simulink model "PMSM_MC_2025a"  (R2025a)
settings: Solver=FixedStepDiscrete  StartTime=0.0  StopTime=10.0  FixedStep=0.00005  RelTol=1e-3
values from neighbouring files (symbols this model uses):
  MC_DCurrLopKi_CFG = 0.008293758    [PMSM_MC_Data_2025a.sldd]
  MC_DCurrLopKp_CFG = 0.0870848    [PMSM_MC_Data_2025a.sldd]
  MC_MotModeDebug_CFG = 255.0    [PMSM_MC_Data_2025a.sldd]
  MC_POLE_NUM_CFG = 7.0    [PMSM_MC_Data_2025a.sldd]
  MC_QCurrLopKi_CFG = 0.008293758    [PMSM_MC_Data_2025a.sldd]
  MC_QCurrLopKp_CFG = 0.0870848    [PMSM_MC_Data_2025a.sldd]
  MC_SpdLopKi_CFG = 1.0E-5    [PMSM_MC_Data_2025a.sldd]
  MC_SpdLopKp_CFG = 0.002    [PMSM_MC_Data_2025a.sldd]
  OpenLoopEn_CFG = 0.0    [PMSM_MC_Data_2025a.sldd]
  SensorLessEn_CFG = 0.0    [PMSM_MC_Data_2025a.sldd]
  SensorLessType_CFG = 1.0    [PMSM_MC_Data_2025a.sldd]
undefined symbols (not defined in the file or in its folder): Ls, magnitude, Rs
libraries: simulink x25, slpidlib x6
(part 2 of 3)

== system PMSM_MC_2025a/PMSM_MC/MC_HighFrqTask/FOC/SVPWM/SevenSegSVPWM ==
  Uα : Inport
  Uβ : Inport  Port=2
  VBus : Inport  Port=3
  Demux : Demux  Outputs=3
  SectorCaculate : Subsystem
  T1T2Caculate : Subsystem
  TcmCaculate : Subsystem
  Tpwm : Constant  Value=single(1)
  XYZCaculate : Subsystem
  UVoltage_PWM : Outport
  VVoltage_PWM : Outport  Port=2
  WVoltage_PWM : Outport  Port=3
  wires:
  Uα/1 -> SectorCaculate/1(Ualpha), XYZCaculate/1(Ualpha)
  Uβ/1 -> XYZCaculate/2(Ubeta), SectorCaculate/2(Ubeta)
  VBus/1 -> XYZCaculate/3(Udc)
  Tpwm/1 -> TcmCaculate/4(Tpwm), T1T2Caculate/3(Tpwm), XYZCaculate/4(Ts)
  SectorCaculate/1(N) -> TcmCaculate/1(N), T1T2Caculate/1(N)
  XYZCaculate/1(XYZ) -> T1T2Caculate/2(XYZ)
  T1T2Caculate/1(T1) -> TcmCaculate/2(T1)
  T1T2Caculate/2(T2) -> TcmCaculate/3(T2)
  TcmCaculate/1(Tcm1 Tcm2 Tcm3) -> Demux/1
  Demux/1 -> UVoltage_PWM/1
  Demux/2 -> VVoltage_PWM/1
  Demux/3 -> WVoltage_PWM/1

== system PMSM_MC_2025a/PMSM_MC/MC_HighFrqTask/FOC/SensorLessAlgorithm/FluxObs+PLL ==
  MotorSpdRef : Inport
  Ialpha : Inport  Port=2
  Ibeta : Inport  Port=3
  Ualpha : Inport  Port=4
  Ubeta : Inport  Port=5
  Enable : EnablePort
  FluxObs : Subsystem
  PLL : Subsystem
  Thetae_Est : Outport
  We_Est : Outport  Port=2
  wires:
  Ubeta/1 -> FluxObs/4(Ubeta)
  Ualpha/1 -> FluxObs/3(Ualpha)
  Ialpha/1 -> FluxObs/1(Ialpha)
  Ibeta/1 -> FluxObs/2(Ibeta)
  PLL/1(Thetae_Est) -> Thetae_Est/1
  PLL/2(We_Est) -> We_Est/1
  FluxObs/2(Flux_beta) -> PLL/3(Flux_beta)
  FluxObs/1(Flux_alpha) -> PLL/2(Flux_alpha)
  MotorSpdRef/1 -> PLL/1(MotorSpdRef)

== system PMSM_MC_2025a/PMSM_MC/MC_HighFrqTask/FOC/SensorLessAlgorithm/Luenberger+PLL ==
  MotorSpdRef : Inport
  Ialpha : Inport  Port=2
  Ibeta : Inport  Port=3
  Ualpha : Inport  Port=4
  Ubeta : Inport  Port=5
  Enable : EnablePort
  Delay : Delay  DelayLength=1
  Luenberger : Subsystem
  PLL : Subsystem
  Thetae_Est : Outport
  We_Est : Outport  Port=2
  wires:
  MotorSpdRef/1 -> PLL/1(MotorSpdRef)
  Luenberger/1(AlphaE) -> PLL/2(AlphaE)
  Luenberger/2(BetaE) -> PLL/3(BetaE)
  PLL/2(We_Est) -> Delay/1, We_Est/1
  PLL/1(Thetae_Est) -> Thetae_Est/1
  Ibeta/1 -> Luenberger/2(Ibeta)
  Ialpha/1 -> Luenberger/1(Ialpha)
  Ualpha/1 -> Luenberger/3(Ualpha)
  Ubeta/1 -> Luenberger/4(Ubeta)
  Delay/1 -> Luenberger/5(We)

== system PMSM_MC_2025a/PMSM_MC/MC_HighFrqTask/FOC/SensorLessAlgorithm/SMO+PLL ==
  MotorSpdRef : Inport
  Ialpha : Inport  Port=2
  Ibeta : Inport  Port=3
  Ualpha : Inport  Port=4
  Ubeta : Inport  Port=5
  Enable : EnablePort
  PLL : Subsystem
  SMO : Subsystem
  Thetae_Est : Outport
  We_Est : Outport  Port=2
  wires:
  MotorSpdRef/1 -> PLL/1(MotorSpdRef)
  SMO/1(AlphaE) -> PLL/2(AlphaE)
  SMO/2(BetaE) -> PLL/3(BetaE)
  PLL/2(We_Est) -> We_Est/1
  PLL/1(Thetae_Est) -> Thetae_Est/1
  Ibeta/1 -> SMO/2(Ibeta)
  Ialpha/1 -> SMO/1(Ialpha)
  Ualpha/1 -> SMO/3(Ualpha)
  Ubeta/1 -> SMO/4(Ubeta)

== system PMSM_MC_2025a/PMSM_MC/MC_HighFrqTask/FOC/SVPWM/SevenSegSVPWM/SectorCaculate ==
  Ualpha : Inport
  Ubeta : Inport  Port=2
  A : Fcn  Expr=u[2]
  Add : Sum  Inputs=+++
  B : Fcn  Expr=u(1)*sqrt(3/4)-0.5*u[2]
  C : Fcn  Expr=-u[1]*sqrt(3/4)-u[2]*0.5
  Constant : Constant  Value=uint8(1)
  Constant1 : Constant  Value=uint8(0)
  Data Type Conversion : DataTypeConversion  OutDataTypeStr=uint8  SaturateOnIntegerOverflow=off  RndMeth=Floor
  Gain : Gain  Gain=2
  Gain1 : Gain  Gain=4
  Mux : Mux  Inputs=2
  Switch : Switch  Criteria=u2 > Threshold  SaturateOnIntegerOverflow=off  InputSameDT=off
  Switch1 : Switch  Criteria=u2 > Threshold  SaturateOnIntegerOverflow=off  InputSameDT=off
  Switch2 : Switch  Criteria=u2 > Threshold  SaturateOnIntegerOverflow=off  InputSameDT=off
  N : Outport
  wires:
  Ualpha/1 -> Mux/1
  Ubeta/1 -> Mux/2
  Mux/1 -> C/1, A/1, B/1
  A/1 -> Switch/2
  B/1 -> Switch1/2
  C/1 -> Switch2/2
  Constant/1 -> Switch/1, Switch2/1, Switch1/1
  Constant1/1 -> Switch/3, Switch1/3, Switch2/3
  Switch2/1 -> Gain1/1
  Switch1/1 -> Gain/1
  Gain/1 -> Add/2
  Gain1/1 -> Add/3
  Switch/1 -> Add/1
  Add/1 -> Data Type Conversion/1
  Data Type Conversion/1 -> N/1

== system PMSM_MC_2025a/PMSM_MC/MC_HighFrqTask/FOC/SVPWM/SevenSegSVPWM/T1T2Caculate ==
  N : Inport
  XYZ : Inport  Port=2
  Tpwm : Inport  Port=3
  Abs : Abs  SaturateOnIntegerOverflow=off
  Abs1 : Abs  SaturateOnIntegerOverflow=off
  Demux : Demux  Outputs=3
  Fcn : Fcn  Expr=u(1)*u(3)/(u(1)+u(2))
  Fcn1 : Fcn  Expr=u(2)*u(3)/(u(1)+u(2))
  Fcn2 : Fcn  Expr=u(3)-u(2)-u(1)
  Gain : Gain  Gain=-1
  Gain1 : Gain  Gain=-1
  Gain2 : Gain  Gain=-1
  Multiport Switch : MultiPortSwitch  Inputs=6  DiagnosticForDefault=None  SaturateOnIntegerOverflow=off  InputSameDT=off
  Multiport Switch1 : MultiPortSwitch  Inputs=6  DiagnosticForDefault=None  SaturateOnIntegerOverflow=off  InputSameDT=off
  Mux : Mux  Inputs=3
  Switch : Switch  SaturateOnIntegerOverflow=off  InputSameDT=off
  Switch1 : Switch  SaturateOnIntegerOverflow=off  InputSameDT=off
  T1 : Outport
  T2 : Outport  Port=2
  wires:
  N/1 -> Multiport Switch/1, Multiport Switch1/1
  XYZ/1 -> Demux/1
  Demux/1 -> Gain/1, Multiport Switch/6, Multiport Switch1/4
  Demux/2 -> Gain1/1, Multiport Switch/3, Multiport Switch1/2
  Demux/3 -> Gain2/1, Multiport Switch1/5, Multiport Switch/2
  Gain/1 -> Multiport Switch1/3, Multiport Switch/5
  Gain2/1 -> Multiport Switch1/7, Multiport Switch/4
  Gain1/1 -> Multiport Switch/7, Multiport Switch1/6
  Multiport Switch/1 -> Switch/1, Mux/1  "T1"
  Multiport Switch1/1 -> Switch1/1, Mux/2  "T2"
  Tpwm/1 -> Mux/3
  Mux/1 -> Fcn1/1, Fcn/1, Fcn2/1
  Fcn/1 -> Switch/3
  Fcn1/1 -> Switch1/3
  Fcn2/1 -> Switch1/2, Switch/2
  Switch/1 -> Abs/1
  Abs/1 -> T1/1
  Switch1/1 -> Abs1/1
  Abs1/1 -> T2/1

== system PMSM_MC_2025a/PMSM_MC/MC_HighFrqTask/FOC/SVPWM/SevenSegSVPWM/TcmCaculate ==
  N : Inport
  T1 : Inport  Port=2
  T2 : Inport  Port=3
  Tpwm : Inport  Port=4
  Fcn : Fcn  Expr=(u(3)+u(1)+u(2))/2
  Fcn1 : Fcn  Expr=(u(3)-u(1)+u(2))/2
  Fcn2 : Fcn  Expr=(u(3)-u(1)-u(2))/2
  Multiport Switch : MultiPortSwitch  Inputs=6  DiagnosticForDefault=None  SaturateOnIntegerOverflow=off  InputSameDT=off
  Multiport Switch1 : MultiPortSwitch  Inputs=6  DiagnosticForDefault=None  SaturateOnIntegerOverflow=off  InputSameDT=off
  Multiport Switch2 : MultiPortSwitch  Inputs=6  DiagnosticForDefault=None  SaturateOnIntegerOverflow=off  InputSameDT=off
  Mux : Mux  Inputs=3
  Mux1 : Mux  Inputs=3
  Tcm1 Tcm2 Tcm3 : Outport
  wires:
  Mux/1 -> Tcm1 Tcm2 Tcm3/1
  T2/1 -> Mux1/2
  T1/1 -> Mux1/1
  Tpwm/1 -> Mux1/3
  Mux1/1 -> Fcn/1, Fcn2/1, Fcn1/1
  N/1 -> Multiport Switch2/1, Multiport Switch1/1, Multiport Switch/1
  Fcn1/1 -> Multiport Switch1/4, Multiport Switch/7, Multiport Switch/2, Multiport Switch1/5, Multiport Switch2/6, Multiport Switch2/3
  Fcn/1 -> Multiport Switch1/6, Multiport Switch2/7, Multiport Switch2/5, Multiport Switch/4, Multiport Switch/3, Multiport Switch1/2
  Fcn2/1 -> Multiport Switch1/7, Multiport Switch/6, Multiport Switch/5, Multiport Switch1/3, Multiport Switch2/4, Multiport Switch2/2
  Multiport Switch/1 -> Mux/1
  Multiport Switch1/1 -> Mux/2
  Multiport Switch2/1 -> Mux/3

== system PMSM_MC_2025a/PMSM_MC/MC_HighFrqTask/FOC/SVPWM/SevenSegSVPWM/XYZCaculate ==
  Ualpha : Inport
  Ubeta : Inport  Port=2
  Udc : Inport  Port=3
  Ts : Inport  Port=4
  Add : Sum
  Add1 : Sum  Inputs=+-
  Fcn : Fcn  Expr=1/u
  Gain : Gain  Gain=3/2
  Gain1 : Gain  Gain=sqrt(3)
  Gain2 : Gain  Gain=sqrt(3)/2
  Mux : Mux  Inputs=3
  Product{,1..3} (4 alike) : Product
  XYZ : Outport
  wires:
  Ualpha/1 -> Gain/1
  Ubeta/1 -> Gain2/1, Gain1/1
  Gain/1 -> Add/2, Add1/2
  Gain1/1 -> Product/1
  Gain2/1 -> Add1/1, Add/1
  Ts/1 -> Product3/1
  Product3/1 -> Product1/2, Product/2, Product2/2
  Add/1 -> Product1/1
  Udc/1 -> Fcn/1
  Fcn/1 -> Product3/2
  Add1/1 -> Product2/1
  Product1/1 -> Mux/2
  Product2/1 -> Mux/3
  Product/1 -> Mux/1
  Mux/1 -> XYZ/1

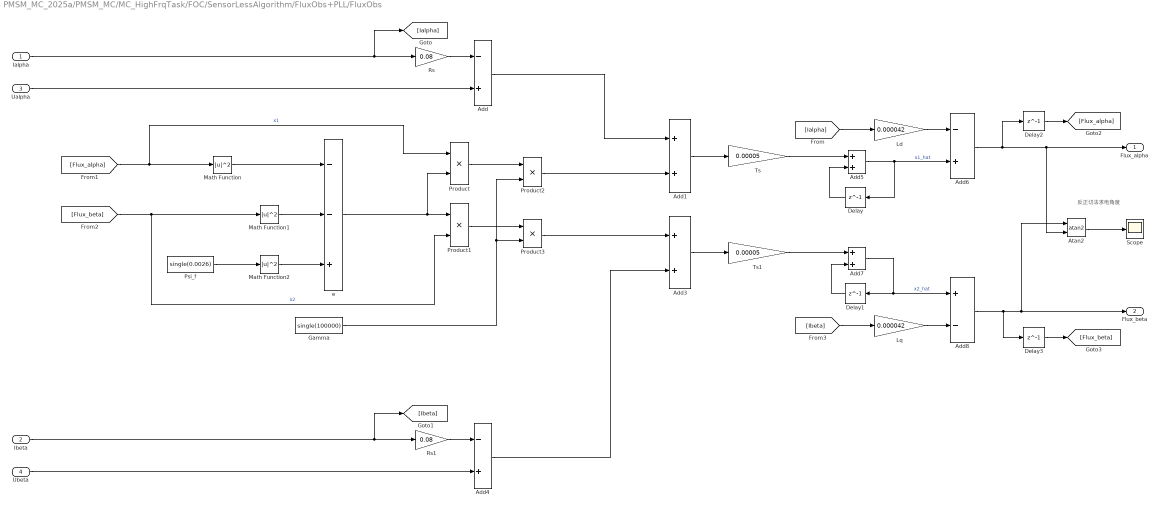
== system PMSM_MC_2025a/PMSM_MC/MC_HighFrqTask/FOC/SensorLessAlgorithm/FluxObs+PLL/FluxObs ==
  note: 反正切法求电角度
  Ialpha : Inport
  Ibeta : Inport  Port=2
  Ualpha : Inport  Port=3
  Ubeta : Inport  Port=4
  Add : Sum  Inputs=-+
  Add{1,3,5,7} (4 alike) : Sum
  Add4 : Sum  Inputs=-+
  Add6 : Sum  Inputs=-+
  Add8 : Sum  Inputs=+-
  Atan2 : Trigonometry  Operator=atan2
  Delay{,1..3} (4 alike) : Delay  DelayLength=1
  Gamma : Constant  Value=single(100000)
  Ld : Gain  Gain=0.000042
  Lq : Gain  Gain=0.000042
  Math Function : Math  Operator=magnitude^2
  Math Function1 : Math  Operator=magnitude^2
  Math Function2 : Math  Operator=magnitude^2
  Product{,1..3} (4 alike) : Product
  Psi_f : Constant  Value=single(0.0026)
  Rs : Gain  Gain=0.08
  Rs1 : Gain  Gain=0.08
  Scope : Scope
      settings: ActiveDisplayYMinimum=-3.9256648123264313  ActiveDisplayYMaximum=3.9258014261722565  DataLoggingVariableName=ScopeData8
  Ts : Gain  Gain=0.00005
  Ts1 : Gain  Gain=0.00005
  e : Sum  Inputs=--+
  Flux_alpha : Outport
  Flux_beta : Outport  Port=2
  wires:
  Ialpha/1 -> [Ialpha], Rs/1
  Rs/1 -> Add/1
  Ualpha/1 -> Add/2
  Add/1 -> Add1/1
  [Flux_alpha] -> Product/1, Math Function/1  "x1"
  Math Function/1 -> e/1
  [Flux_beta] -> Product1/2, Math Function1/1  "x2"
  Math Function1/1 -> e/2
  Math Function2/1 -> e/3
  Psi_f/1 -> Math Function2/1
  e/1 -> Product1/1, Product/2
  Product/1 -> Product2/1
  Product1/1 -> Product3/1
  Gamma/1 -> Product2/2, Product3/2
  Product2/1 -> Add1/2
  Product3/1 -> Add3/1
  Ubeta/1 -> Add4/2
  Ibeta/1 -> [Ibeta], Rs1/1
  Rs1/1 -> Add4/1
  Add4/1 -> Add3/2
  Add1/1 -> Ts/1
  Add3/1 -> Ts1/1
  Ts/1 -> Add5/1
  [Ialpha] -> Ld/1
  Ld/1 -> Add6/1
  Add5/1 -> Delay/1, Add6/2  "x1_hat"
  Delay/1 -> Add5/2
  Ts1/1 -> Add7/1
  Add7/1 -> Add8/1, Delay1/1  "x2_hat"
  Delay1/1 -> Add7/2
  Lq/1 -> Add8/2
  [Ibeta] -> Lq/1
  Add6/1 -> Delay2/1, Atan2/2, Flux_alpha/1
  Add8/1 -> Delay3/1, Atan2/1, Flux_beta/1
  Delay2/1 -> [Flux_alpha]
  Delay3/1 -> [Flux_beta]
  Atan2/1 -> Scope/1

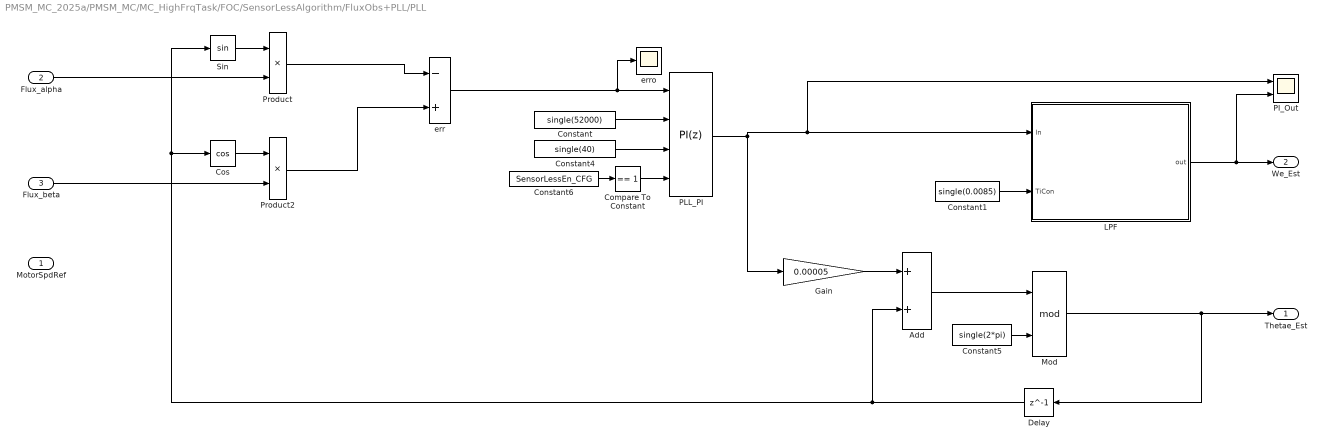
== system PMSM_MC_2025a/PMSM_MC/MC_HighFrqTask/FOC/SensorLessAlgorithm/FluxObs+PLL/PLL ==
  MotorSpdRef : Inport
  Flux_alpha : Inport  Port=2
  Flux_beta : Inport  Port=3
  Add : Sum
  Compare To Constant : simulink/Logic and Bit Operations/Compare To Constant  relop===  const=1  OutDataTypeStr=boolean
  Constant : Constant  Value=single(52000)
  Constant1 : Constant  Value=single(0.0085)
  Constant4 : Constant  Value=single(40)
  Constant5 : Constant  Value=single(2*pi)
  Constant6 : Constant  Value=SensorLessEn_CFG
  Cos : Trigonometry  Operator=cos
  Delay : Delay  DelayLength=1
  Gain : Gain  Gain=0.00005
  LPF : Subsystem
  Mod : Math  Operator=mod
  PI_Out : Scope  NumInputPorts=2
      settings: ActiveDisplayYMinimum=-82.912358522415147  ActiveDisplayYMaximum=519.20902562141418  DataLoggingVariableName=ScopeData11
  PLL_PI : slpidlib/PID Controller  Controller=PI  Form=Parallel  TimeDomain=Discrete-time  UseExternalTs=off  SampleTime=-1  IntegratorMethod=Forward Euler  FilterMethod=Forward Euler  ControllerParametersSource=external  P=1  I=1  UseKiTs=on  D=0  UseExternalDerivativeSource=off  N=100  UseFilter=on  TunerSelectOption=Transfer Function Based (PID Tuner App)  InitialConditionSource=internal  InitialConditionForIntegrator=0  InitialConditionForFilter=0  DifferentiatorICPrevScaledInput=0  ExternalReset=rising  TrackingMode=off  Kt=1  LimitOutput=off  SatLimitsSource=internal  UpperSaturationLimit=inf  LowerSaturationLimit=-inf  LinearizeAsGain=off  AntiWindupMode=none  Kb=1  LimitIntegrator=off  UpperIntegratorSaturationLimit=8000  LowerIntegratorSaturationLimit=-8000  POutMin=[]  POutMax=[]  IOutMin=[]  IOutMax=[]  DOutMin=[]  DOutMax=[]  NOutMin=[]  NOutMax=[]  SumOutMin=[]  SumOutMax=[]  SaturationOutMin=[]  SaturationOutMax=[]  PParamMin=[]  PParamMax=[]  IParamMin=[]  IParamMax=[]  DParamMin=[]  DParamMax=[]  NParamMin=[]  NParamMax=[]  KbParamMin=[]  KbParamMax=[]  KtParamMin=[]  KtParamMax=[]  KbOutMin=[]  KbOutMax=[]  KtOutMin=[]  KtOutMax=[]  IntegratorOutMin=[]  IntegratorOutMax=[]  FilterOutMin=[]  FilterOutMax=[]  SumI1OutMin=[]  SumI1OutMax=[]  SumI2OutMin=[]  SumI2OutMax=[]  SumI3OutMin=[]  SumI3OutMax=[]  SumI4OutMin=[]  SumI4OutMax=[]  SumDOutMin=[]  SumDOutMax=[]  DifferentiatorOutMin=[]  DifferentiatorOutMax=[]  FilterDiffOutCoefMin=[]  FilterDiffOutCoefMax=[]  ReciprocalOutMin=[]  ReciprocalOutMax=[]  SumDenOutMin=[]  SumDenOutMax=[]  SumNumOutMin=[]  SumNumOutMax=[]  DivideOutMin=[]  DivideOutMax=[]  UdiffTsProdOutMin=[]  UdiffTsProdOutMax=[]  NTsProdOutMin=[]  NTsProdOutMax=[]  UintegralTsProdOutMin=[]  UintegralTsProdOutMax=[]  UngainTsProdOutMin=[]  UngainTsProdOutMax=[]  ClampingZeroOutDataTypeStr=Inherit: Inherit via back propagation  ClampingZeroOutMin=[]  ClampingZeroOutMax=[]  FilterDenConstantOutDataTypeStr=Inherit: Inherit via back propagation  FilterDenConstantOutMin=[]  FilterDenConstantOutMax=[]  PCopyOutDataTypeStr=Inherit: Inherit via back propagation  PCopyOutMin=[]  PCopyOutMax=[]  NCopyOutDataTypeStr=Inherit: Inherit via back propagation  NCopyOutMin=[]  NCopyOutMax=[]  IntegratorContinuousStateAttributes=''  IntegratorStateMustResolveToSignalObject=off  IntegratorRTWStateStorageClass=Auto  FilterContinuousStateAttributes=''  FilterStateMustResolveToSignalObject=off  FilterRTWStateStorageClass=Auto  ParallelPVariant=ExternalParameters  IdealPVariant=Disabled  IVariant=ExternalParameters  DVariant=Disabled  IntegratorVariant=Discrete  SatVariant=Disabled  AWVariant=Passthrough  PCopyVariant=Disabled  TRVariant=Disabled  FdbkBlocksVariant=Forward  IdealPFdbkVariant=Disabled  SatFdbkVariant=Disabled  DerivativeFilterVariant=Disabled  NVariant=Disabled  NCopyVariant=Disabled_SignalSpec  FilterICVariant=Disabled  IntegratorICVariant=InternalICs  ExternalResetVariant=ExternalReset  TRSumVariant=Passthrough  SumFdbkVariant=Disabled  SumVariant=Sum_PI  TsampFilterVariant=InternalTs  TsampNgainVariant=Passthrough  TsampIntegralVariant=Disabled_SignalSpec  ExternalSaturationOutDataTypeStr=Inherit: Same as second input  DerivativeSourceVariant=Disabled  PreIntVariant=InternalPreInt
      settings: LibrarySourceBlock=simulink/Discrete/Discrete PID Controller
  Product : Product
  Product2 : Product
  Sin : Trigonometry
  err : Sum  Inputs=-+
  erro : Scope
      settings: ActiveDisplayYMinimum=-0.010186117957346141  ActiveDisplayYMaximum=0.0015268082497641442  DataLoggingVariableName=ScopeData10
  Thetae_Est : Outport
  We_Est : Outport  Port=2
  wires:
  Delay/1 -> Add/2, Cos/1, Sin/1
  Mod/1 -> Thetae_Est/1, Delay/1
  Constant5/1 -> Mod/2
  Add/1 -> Mod/1
  Gain/1 -> Add/1
  PLL_PI/1 -> PI_Out/1, LPF/1(In), Gain/1
  Constant4/1 -> PLL_PI/3
  Constant/1 -> PLL_PI/2
  Cos/1 -> Product2/1
  Sin/1 -> Product/1
  LPF/1(out) -> PI_Out/2, We_Est/1
  Constant1/1 -> LPF/2(TiCon)
  Flux_alpha/1 -> Product/2
  Flux_beta/1 -> Product2/2
  Product/1 -> err/1
  Product2/1 -> err/2
  err/1 -> erro/1, PLL_PI/1
  Constant6/1 -> Compare To Constant/1
  Compare To Constant/1 -> PLL_PI/4

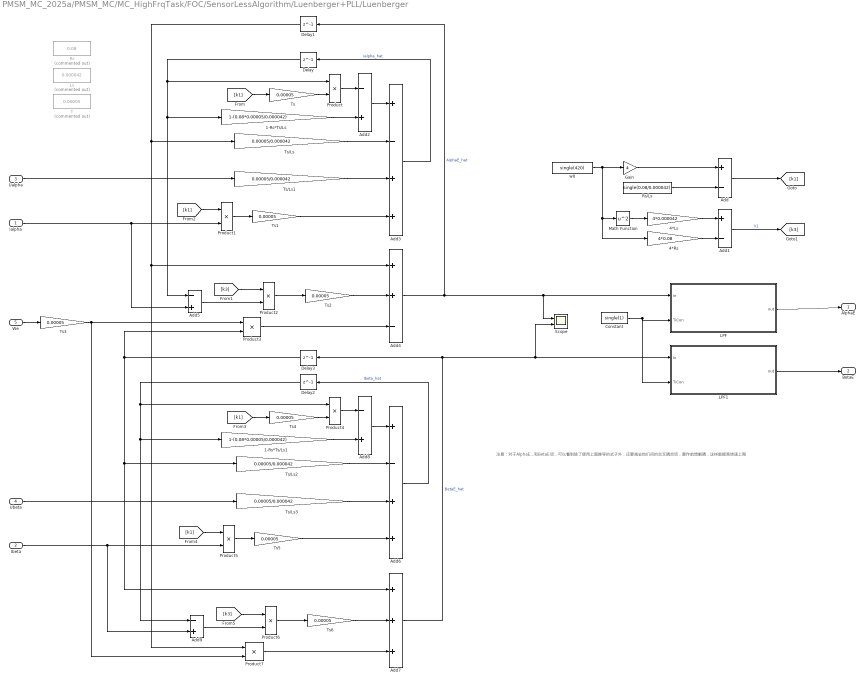
== system PMSM_MC_2025a/PMSM_MC/MC_HighFrqTask/FOC/SensorLessAlgorithm/Luenberger+PLL/Luenberger ==
  note: 注意：对于AlphaE和BetaE项，可以看到除了使用上面推导的式子外，还要减去他们间的交叉耦合项，算作前馈解耦，这样能提高转速上限
  Ialpha : Inport
  Ibeta : Inport  Port=2
  Ualpha : Inport  Port=3
  Ubeta : Inport  Port=4
  We : Inport  Port=5
  1-Rs*Ts/Ls : Gain  Gain=1-(0.08*0.00005/0.000042)
  1-Rs*Ts/Ls1 : Gain  Gain=1-(0.08*0.00005/0.000042)
  4*Ls : Gain  Gain=4*0.000042
  4*Rs : Gain  Gain=4*0.08
  Add : Sum  Inputs=+-
  Add1 : Sum  Inputs=+-
  Add{2,5,8..9} (4 alike) : Sum  Inputs=-+
  Add3 : Sum  Inputs=+-++
  Add4 : Sum  Inputs=++-
  Add6 : Sum  Inputs=+-++
  Add7 : Sum  Inputs=+++
  Constant : Constant  Value=single(1)
  Delay{,1..3} (4 alike) : Delay  DelayLength=1
  Gain : Gain  Gain=4
  LPF : Subsystem
  LPF1 : Subsystem
  Ls : Constant  Commented=on  Value=0.000042
  Math Function : Math  Operator=square
  Product{,1..7} (8 alike) : Product
  Rs : Constant  Commented=on  Value=0.08
  Rs/Ls : Constant  Value=single(0.08/0.000042)
  Scope : Scope  NumInputPorts=2
      settings: ActiveDisplayYMinimum=-21.479682207107544  ActiveDisplayYMaximum=21.825211763381958  DataLoggingVariableName=ScopeData18
  T : Constant  Commented=on  Value=0.00005
  Ts{,1..6} (7 alike) : Gain  Gain=0.00005
  Ts/Ls{,1..3} (4 alike) : Gain  Gain=0.00005/0.000042
  w0 : Constant  Value=single(420)
  AlphaE : Outport
  BetaE : Outport  Port=2
  wires:
  w0/1 -> 4*Rs/1, Math Function/1, Gain/1
  Add/1 -> [k1]
  Rs/Ls/1 -> Add/2
  Gain/1 -> Add/1
  4*Ls/1 -> Add1/1
  4*Rs/1 -> Add1/2
  Math Function/1 -> 4*Ls/1
  Add1/1 -> [k3]  "k1"
  [k1] -> Ts/1
  Ts/1 -> Product/2
  Product/1 -> Add2/1
  1-Rs*Ts/Ls/1 -> Add2/2
  Ts/Ls/1 -> Add3/2
  Add2/1 -> Add3/1
  Ts/Ls1/1 -> Add3/3
  [k1] -> Product1/1
  Product1/1 -> Ts1/1
  Ts1/1 -> Add3/4
  Ialpha/1 -> Add5/2, Product1/2
  Ualpha/1 -> Ts/Ls1/1
  Add3/1 -> Delay/1  "Ialpha_hat"
  Delay/1 -> Add5/1, 1-Rs*Ts/Ls/1, Product/1
  Add4/1 -> Scope/1, LPF/1(In), Delay1/1  "AlphaE_hat"
  Delay1/1 -> Product7/1, Add4/1, Ts/Ls/1
  Ts2/1 -> Add4/2
  Product2/1 -> Ts2/1
  [k3] -> Product2/1
  Add5/1 -> Product2/2
  Constant/1 -> LPF1/2(TiCon), LPF/2(TiCon)
  LPF1/1(out) -> BetaE/1
  LPF/1(out) -> AlphaE/1
  We/1 -> Ts3/1
  Product3/1 -> Add4/3
  Add6/1 -> Delay2/1  "Ibeta_hat"
  Product4/1 -> Add8/1
  Delay2/1 -> Product4/1, 1-Rs*Ts/Ls1/1, Add9/1
  1-Rs*Ts/Ls1/1 -> Add8/2
  Ts4/1 -> Product4/2
  [k1] -> Ts4/1
  Add8/1 -> Add6/1
  [k1] -> Product5/1
  Ibeta/1 -> Product5/2, Add9/2
  Delay3/1 -> Ts/Ls2/1, Add7/1, Product3/2
  Ubeta/1 -> Ts/Ls3/1
  Product5/1 -> Ts5/1
  Ts/Ls3/1 -> Add6/3
  Ts5/1 -> Add6/4
  Ts/Ls2/1 -> Add6/2
  Product7/1 -> Add7/3
  Product6/1 -> Ts6/1
  [k3] -> Product6/1
  Add9/1 -> Product6/2
  Ts3/1 -> Product3/1, Product7/2
  Ts6/1 -> Add7/2
  Add7/1 -> Scope/2, LPF1/1(In), Delay3/1  "BetaE_hat"

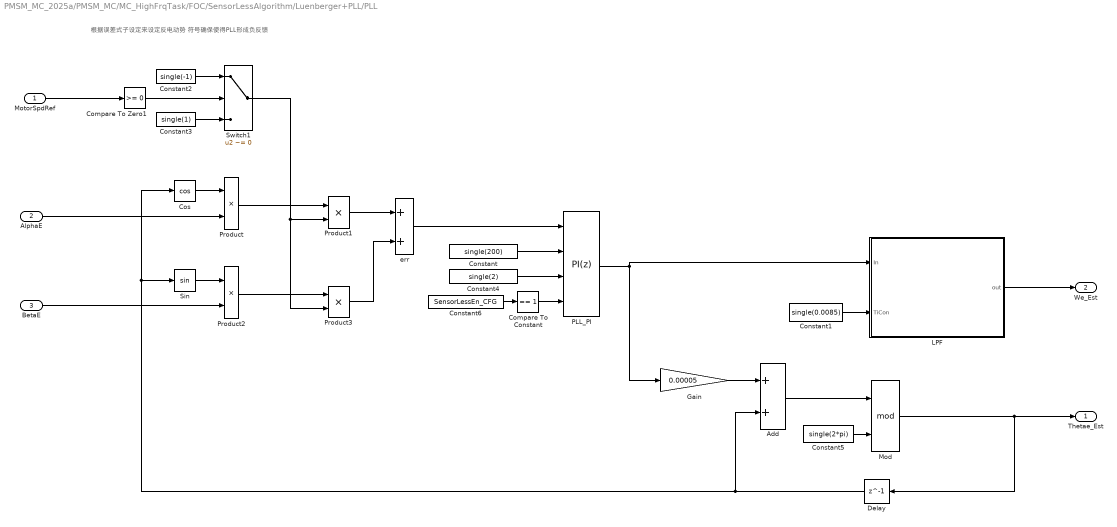
== system PMSM_MC_2025a/PMSM_MC/MC_HighFrqTask/FOC/SensorLessAlgorithm/Luenberger+PLL/PLL ==
  note: 根据误差式子设定来设定反电动势
      | 符号确保使得PLL形成负反馈
  MotorSpdRef : Inport
  AlphaE : Inport  Port=2
  BetaE : Inport  Port=3
  Add : Sum
  Compare To Constant : simulink/Logic and Bit Operations/Compare To Constant  relop===  const=1  OutDataTypeStr=boolean
  Compare To Zero1 : simulink/Logic and Bit Operations/Compare To Zero  relop=>=  OutDataTypeStr=boolean
  Constant : Constant  Value=single(200)
  Constant1 : Constant  Value=single(0.0085)
  Constant2 : Constant  Value=single(-1)
  Constant3 : Constant  Value=single(1)
  Constant4 : Constant  Value=single(2)
  Constant5 : Constant  Value=single(2*pi)
  Constant6 : Constant  Value=SensorLessEn_CFG
  Cos : Trigonometry  Operator=cos
  Delay : Delay  DelayLength=1
  Gain : Gain  Gain=0.00005
  LPF : Subsystem
  Mod : Math  Operator=mod
  PLL_PI : slpidlib/PID Controller  Controller=PI  Form=Parallel  TimeDomain=Discrete-time  UseExternalTs=off  SampleTime=-1  IntegratorMethod=Forward Euler  FilterMethod=Forward Euler  ControllerParametersSource=external  P=1  I=1  UseKiTs=on  D=0  UseExternalDerivativeSource=off  N=100  UseFilter=on  TunerSelectOption=Transfer Function Based (PID Tuner App)  InitialConditionSource=internal  InitialConditionForIntegrator=0  InitialConditionForFilter=0  DifferentiatorICPrevScaledInput=0  ExternalReset=rising  TrackingMode=off  Kt=1  LimitOutput=off  SatLimitsSource=internal  UpperSaturationLimit=inf  LowerSaturationLimit=-inf  LinearizeAsGain=off  AntiWindupMode=none  Kb=1  LimitIntegrator=off  UpperIntegratorSaturationLimit=inf  LowerIntegratorSaturationLimit=-inf  POutMin=[]  POutMax=[]  IOutMin=[]  IOutMax=[]  DOutMin=[]  DOutMax=[]  NOutMin=[]  NOutMax=[]  SumOutMin=[]  SumOutMax=[]  SaturationOutMin=[]  SaturationOutMax=[]  PParamMin=[]  PParamMax=[]  IParamMin=[]  IParamMax=[]  DParamMin=[]  DParamMax=[]  NParamMin=[]  NParamMax=[]  KbParamMin=[]  KbParamMax=[]  KtParamMin=[]  KtParamMax=[]  KbOutMin=[]  KbOutMax=[]  KtOutMin=[]  KtOutMax=[]  IntegratorOutMin=[]  IntegratorOutMax=[]  FilterOutMin=[]  FilterOutMax=[]  SumI1OutMin=[]  SumI1OutMax=[]  SumI2OutMin=[]  SumI2OutMax=[]  SumI3OutMin=[]  SumI3OutMax=[]  SumI4OutMin=[]  SumI4OutMax=[]  SumDOutMin=[]  SumDOutMax=[]  DifferentiatorOutMin=[]  DifferentiatorOutMax=[]  FilterDiffOutCoefMin=[]  FilterDiffOutCoefMax=[]  ReciprocalOutMin=[]  ReciprocalOutMax=[]  SumDenOutMin=[]  SumDenOutMax=[]  SumNumOutMin=[]  SumNumOutMax=[]  DivideOutMin=[]  DivideOutMax=[]  UdiffTsProdOutMin=[]  UdiffTsProdOutMax=[]  NTsProdOutMin=[]  NTsProdOutMax=[]  UintegralTsProdOutMin=[]  UintegralTsProdOutMax=[]  UngainTsProdOutMin=[]  UngainTsProdOutMax=[]  ClampingZeroOutDataTypeStr=Inherit: Inherit via back propagation  ClampingZeroOutMin=[]  ClampingZeroOutMax=[]  FilterDenConstantOutDataTypeStr=Inherit: Inherit via back propagation  FilterDenConstantOutMin=[]  FilterDenConstantOutMax=[]  PCopyOutDataTypeStr=Inherit: Inherit via back propagation  PCopyOutMin=[]  PCopyOutMax=[]  NCopyOutDataTypeStr=Inherit: Inherit via back propagation  NCopyOutMin=[]  NCopyOutMax=[]  IntegratorContinuousStateAttributes=''  IntegratorStateMustResolveToSignalObject=off  IntegratorRTWStateStorageClass=Auto  FilterContinuousStateAttributes=''  FilterStateMustResolveToSignalObject=off  FilterRTWStateStorageClass=Auto  ParallelPVariant=ExternalParameters  IdealPVariant=Disabled  IVariant=ExternalParameters  DVariant=Disabled  IntegratorVariant=Discrete  SatVariant=Disabled  AWVariant=Passthrough  PCopyVariant=Disabled  TRVariant=Disabled  FdbkBlocksVariant=Forward  IdealPFdbkVariant=Disabled  SatFdbkVariant=Disabled  DerivativeFilterVariant=Disabled  NVariant=Disabled  NCopyVariant=Disabled_SignalSpec  FilterICVariant=Disabled  IntegratorICVariant=InternalICs  ExternalResetVariant=ExternalReset  TRSumVariant=Passthrough  SumFdbkVariant=Disabled  SumVariant=Sum_PI  TsampFilterVariant=InternalTs  TsampNgainVariant=Passthrough  TsampIntegralVariant=Disabled_SignalSpec  ExternalSaturationOutDataTypeStr=Inherit: Same as second input  DerivativeSourceVariant=Disabled  PreIntVariant=InternalPreInt
      settings: LibrarySourceBlock=simulink/Discrete/Discrete PID Controller
  Product{,1..3} (4 alike) : Product
  Sin : Trigonometry
  Switch1 : Switch  Criteria=u2 ~= 0  SaturateOnIntegerOverflow=off  InputSameDT=off
  err : Sum
  Thetae_Est : Outport
  We_Est : Outport  Port=2
  wires:
  Gain/1 -> Add/1
  Mod/1 -> Delay/1, Thetae_Est/1
  AlphaE/1 -> Product/2
  Constant4/1 -> PLL_PI/3
  Product/1 -> Product1/1
  Constant3/1 -> Switch1/3
  Constant5/1 -> Mod/2
  Switch1/1 -> Product3/2, Product1/2
  Product3/1 -> err/2
  Delay/1 -> Cos/1, Sin/1, Add/2
  err/1 -> PLL_PI/1
  Compare To Zero1/1 -> Switch1/2
  Constant2/1 -> Switch1/1
  PLL_PI/1 -> LPF/1(In), Gain/1
  Cos/1 -> Product/1
  Sin/1 -> Product2/1
  MotorSpdRef/1 -> Compare To Zero1/1
  BetaE/1 -> Product2/2
  Constant/1 -> PLL_PI/2
  LPF/1(out) -> We_Est/1
  Product1/1 -> err/1
  Constant1/1 -> LPF/2(TiCon)
  Product2/1 -> Product3/1
  Add/1 -> Mod/1
  Constant6/1 -> Compare To Constant/1
  Compare To Constant/1 -> PLL_PI/4

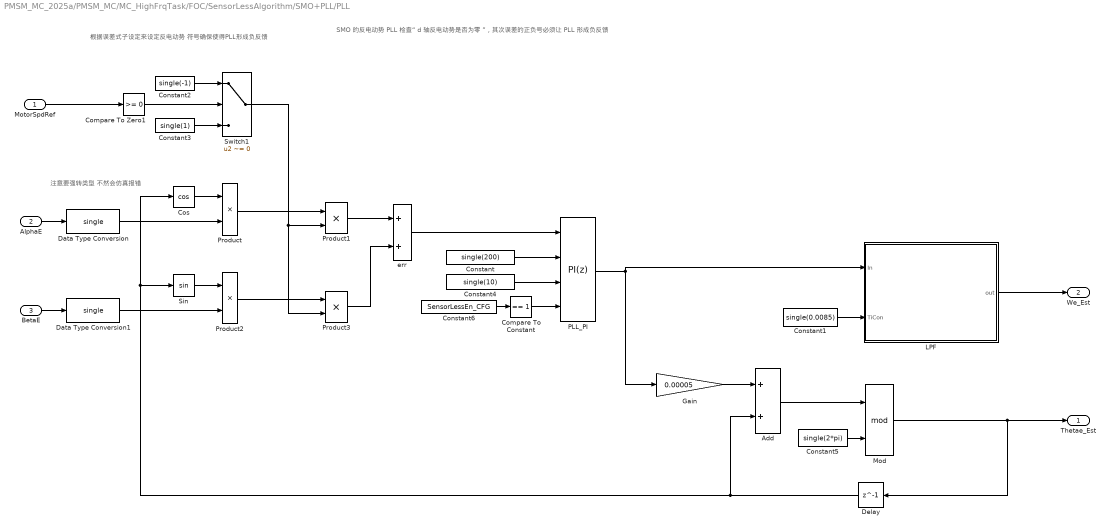
== system PMSM_MC_2025a/PMSM_MC/MC_HighFrqTask/FOC/SensorLessAlgorithm/SMO+PLL/PLL ==
  note: SMO 的反电动势 PLL 检查“ d 轴反电动势是否为零 ”，其次误差的正负号必须让 PLL 形成负反馈
  note: 注意要强转类型
      | 不然会仿真报错
  note: 根据误差式子设定来设定反电动势
      | 符号确保使得PLL形成负反馈
  MotorSpdRef : Inport
  AlphaE : Inport  Port=2
  BetaE : Inport  Port=3
  Add : Sum
  Compare To Constant : simulink/Logic and Bit Operations/Compare To Constant  relop===  const=1  OutDataTypeStr=boolean
  Compare To Zero1 : simulink/Logic and Bit Operations/Compare To Zero  relop=>=  OutDataTypeStr=boolean
  Constant : Constant  Value=single(200)
  Constant1 : Constant  Value=single(0.0085)
  Constant2 : Constant  Value=single(-1)
  Constant3 : Constant  Value=single(1)
  Constant4 : Constant  Value=single(10)
  Constant5 : Constant  Value=single(2*pi)
  Constant6 : Constant  Value=SensorLessEn_CFG
  Cos : Trigonometry  Operator=cos
  Data Type Conversion : DataTypeConversion  OutDataTypeStr=single  SaturateOnIntegerOverflow=off  RndMeth=Floor
  Data Type Conversion1 : DataTypeConversion  OutDataTypeStr=single  SaturateOnIntegerOverflow=off  RndMeth=Floor
  Delay : Delay  DelayLength=1
  Gain : Gain  Gain=0.00005
  LPF : Subsystem
  Mod : Math  Operator=mod
  PLL_PI : slpidlib/PID Controller  Controller=PI  Form=Parallel  TimeDomain=Discrete-time  UseExternalTs=off  SampleTime=-1  IntegratorMethod=Forward Euler  FilterMethod=Forward Euler  ControllerParametersSource=external  P=1  I=1  UseKiTs=on  D=0  UseExternalDerivativeSource=off  N=100  UseFilter=on  TunerSelectOption=Transfer Function Based (PID Tuner App)  InitialConditionSource=internal  InitialConditionForIntegrator=0  InitialConditionForFilter=0  DifferentiatorICPrevScaledInput=0  ExternalReset=rising  TrackingMode=off  Kt=1  LimitOutput=off  SatLimitsSource=internal  UpperSaturationLimit=inf  LowerSaturationLimit=-inf  LinearizeAsGain=off  AntiWindupMode=none  Kb=1  LimitIntegrator=off  UpperIntegratorSaturationLimit=inf  LowerIntegratorSaturationLimit=-inf  POutMin=[]  POutMax=[]  IOutMin=[]  IOutMax=[]  DOutMin=[]  DOutMax=[]  NOutMin=[]  NOutMax=[]  SumOutMin=[]  SumOutMax=[]  SaturationOutMin=[]  SaturationOutMax=[]  PParamMin=[]  PParamMax=[]  IParamMin=[]  IParamMax=[]  DParamMin=[]  DParamMax=[]  NParamMin=[]  NParamMax=[]  KbParamMin=[]  KbParamMax=[]  KtParamMin=[]  KtParamMax=[]  KbOutMin=[]  KbOutMax=[]  KtOutMin=[]  KtOutMax=[]  IntegratorOutMin=[]  IntegratorOutMax=[]  FilterOutMin=[]  FilterOutMax=[]  SumI1OutMin=[]  SumI1OutMax=[]  SumI2OutMin=[]  SumI2OutMax=[]  SumI3OutMin=[]  SumI3OutMax=[]  SumI4OutMin=[]  SumI4OutMax=[]  SumDOutMin=[]  SumDOutMax=[]  DifferentiatorOutMin=[]  DifferentiatorOutMax=[]  FilterDiffOutCoefMin=[]  FilterDiffOutCoefMax=[]  ReciprocalOutMin=[]  ReciprocalOutMax=[]  SumDenOutMin=[]  SumDenOutMax=[]  SumNumOutMin=[]  SumNumOutMax=[]  DivideOutMin=[]  DivideOutMax=[]  UdiffTsProdOutMin=[]  UdiffTsProdOutMax=[]  NTsProdOutMin=[]  NTsProdOutMax=[]  UintegralTsProdOutMin=[]  UintegralTsProdOutMax=[]  UngainTsProdOutMin=[]  UngainTsProdOutMax=[]  ClampingZeroOutDataTypeStr=Inherit: Inherit via back propagation  ClampingZeroOutMin=[]  ClampingZeroOutMax=[]  FilterDenConstantOutDataTypeStr=Inherit: Inherit via back propagation  FilterDenConstantOutMin=[]  FilterDenConstantOutMax=[]  PCopyOutDataTypeStr=Inherit: Inherit via back propagation  PCopyOutMin=[]  PCopyOutMax=[]  NCopyOutDataTypeStr=Inherit: Inherit via back propagation  NCopyOutMin=[]  NCopyOutMax=[]  IntegratorContinuousStateAttributes=''  IntegratorStateMustResolveToSignalObject=off  IntegratorRTWStateStorageClass=Auto  FilterContinuousStateAttributes=''  FilterStateMustResolveToSignalObject=off  FilterRTWStateStorageClass=Auto  ParallelPVariant=ExternalParameters  IdealPVariant=Disabled  IVariant=ExternalParameters  DVariant=Disabled  IntegratorVariant=Discrete  SatVariant=Disabled  AWVariant=Passthrough  PCopyVariant=Disabled  TRVariant=Disabled  FdbkBlocksVariant=Forward  IdealPFdbkVariant=Disabled  SatFdbkVariant=Disabled  DerivativeFilterVariant=Disabled  NVariant=Disabled  NCopyVariant=Disabled_SignalSpec  FilterICVariant=Disabled  IntegratorICVariant=InternalICs  ExternalResetVariant=ExternalReset  TRSumVariant=Passthrough  SumFdbkVariant=Disabled  SumVariant=Sum_PI  TsampFilterVariant=InternalTs  TsampNgainVariant=Passthrough  TsampIntegralVariant=Disabled_SignalSpec  ExternalSaturationOutDataTypeStr=Inherit: Same as second input  DerivativeSourceVariant=Disabled  PreIntVariant=InternalPreInt
      settings: LibrarySourceBlock=simulink/Discrete/Discrete PID Controller
  Product{,1..3} (4 alike) : Product
  Sin : Trigonometry
  Switch1 : Switch  Criteria=u2 ~= 0  SaturateOnIntegerOverflow=off  InputSameDT=off
  err : Sum
  Thetae_Est : Outport
  We_Est : Outport  Port=2
  wires:
  MotorSpdRef/1 -> Compare To Zero1/1
  Compare To Zero1/1 -> Switch1/2
  Constant1/1 -> LPF/2(TiCon)
  LPF/1(out) -> We_Est/1
  Constant2/1 -> Switch1/1
  Constant3/1 -> Switch1/3
  Cos/1 -> Product/1
  Product/1 -> Product1/1
  Switch1/1 -> Product3/2, Product1/2
  Sin/1 -> Product2/1
  Product2/1 -> Product3/1
  Product1/1 -> err/1
  Product3/1 -> err/2
  err/1 -> PLL_PI/1
  Constant/1 -> PLL_PI/2
  Constant4/1 -> PLL_PI/3
  PLL_PI/1 -> LPF/1(In), Gain/1
  Gain/1 -> Add/1
  Add/1 -> Mod/1
  Constant5/1 -> Mod/2
  Mod/1 -> Delay/1, Thetae_Est/1
  Delay/1 -> Cos/1, Sin/1, Add/2
  BetaE/1 -> Data Type Conversion1/1
  AlphaE/1 -> Data Type Conversion/1
  Data Type Conversion/1 -> Product/2
  Data Type Conversion1/1 -> Product2/2
  Constant6/1 -> Compare To Constant/1
  Compare To Constant/1 -> PLL_PI/4

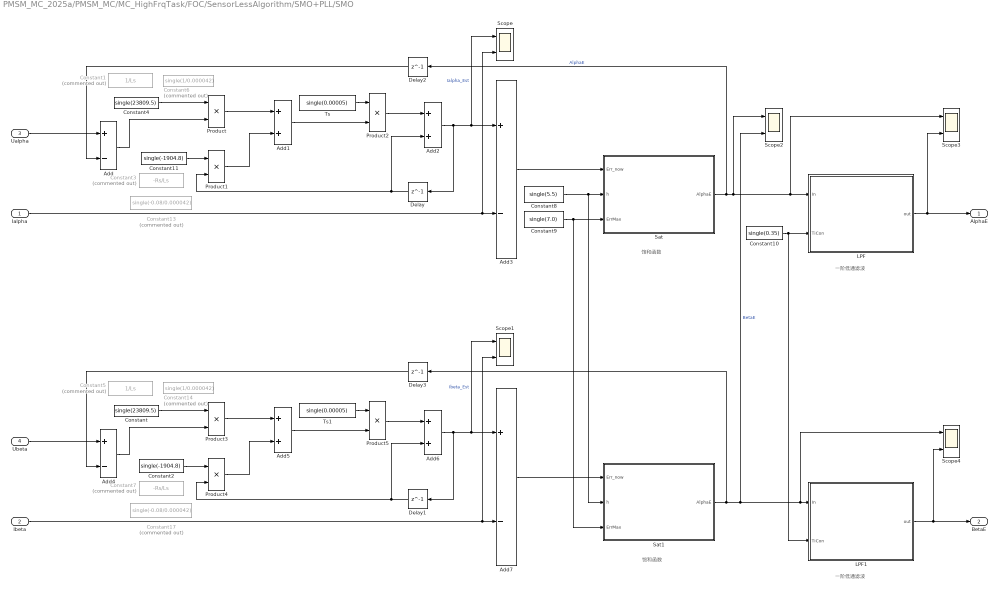
== system PMSM_MC_2025a/PMSM_MC/MC_HighFrqTask/FOC/SensorLessAlgorithm/SMO+PLL/SMO ==
  note: 一阶低通滤波
  note: 饱和函数
  note: 饱和函数
  note: 一阶低通滤波
  Ialpha : Inport
  Ibeta : Inport  Port=2
  Ualpha : Inport  Port=3
  Ubeta : Inport  Port=4
  Add : Sum  Inputs=+-  OutDataTypeStr=single
  Add{1..2,5..6} (4 alike) : Sum
  Add3 : Sum  Inputs=+-  OutDataTypeStr=single
  Add4 : Sum  Inputs=+-
  Add7 : Sum  Inputs=+-
  Constant : Constant  Value=single(23809.5)
  Constant1 : Constant  Commented=on  Value=1/Ls
  Constant10 : Constant  Value=single(0.35)
  Constant11 : Constant  Value=single(-1904.8)
  Constant13 : Constant  Commented=on  Value=single(-0.08/0.000042)
  Constant14 : Constant  Commented=on  Value=single(1/0.000042)
  Constant17 : Constant  Commented=on  Value=single(-0.08/0.000042)
  Constant2 : Constant  Value=single(-1904.8)
  Constant3 : Constant  Commented=on  Value=-Rs/Ls
  Constant4 : Constant  Value=single(23809.5)
  Constant5 : Constant  Commented=on  Value=1/Ls
  Constant6 : Constant  Commented=on  Value=single(1/0.000042)
  Constant7 : Constant  Commented=on  Value=-Rs/Ls
  Constant8 : Constant  Value=single(5.5)
  Constant9 : Constant  Value=single(7.0)
  Delay{,1..3} (4 alike) : Delay  DelayLength=1
  LPF : Subsystem
  LPF1 : Subsystem
  Product{,1..5} (6 alike) : Product
  Sat : Subsystem
  Sat1 : Subsystem
  Scope{,1..4} (5 alike) : Scope  NumInputPorts=2
      Scope settings: ActiveDisplayYMinimum=-11.265603890227075  ActiveDisplayYMaximum=11.401321085088421  DataLoggingVariableName=ScopeData2
      Scope1 settings: DataLoggingVariableName=ScopeData3
      Scope2 settings: ActiveDisplayYMinimum=-6.875  ActiveDisplayYMaximum=6.875  DataLoggingVariableName=ScopeData4
      Scope3 settings: DataLoggingVariableName=ScopeData5
      Scope4 settings: DataLoggingVariableName=ScopeData6
  Ts : Constant  Value=single(0.00005)
  Ts1 : Constant  Value=single(0.00005)
  AlphaE : Outport
  BetaE : Outport  Port=2
  wires:
  Ualpha/1 -> Add/1
  Constant4/1 -> Product/1
  Add/1 -> Product/2
  Product/1 -> Add1/1
  Constant11/1 -> Product1/1
  Product1/1 -> Add1/2
  Add1/1 -> Product2/2
  Ts/1 -> Product2/1
  Product2/1 -> Add2/1
  Add2/1 -> Delay/1, Scope/1, Add3/1  "Ialpha_Est"
  Delay/1 -> Add2/2, Product1/2
  Ialpha/1 -> Scope/2, Add3/2
  Product5/1 -> Add6/1
  Delay1/1 -> Add6/2, Product4/2
  Product3/1 -> Add5/1
  Ibeta/1 -> Scope1/2, Add7/2
  Ts1/1 -> Product5/1
  Add4/1 -> Product3/2
  Constant/1 -> Product3/1
  Product4/1 -> Add5/2
  Constant2/1 -> Product4/1
  Add5/1 -> Product5/2
  Add6/1 -> Delay1/1, Scope1/1, Add7/1  "Ibeta_Est"
  Ubeta/1 -> Add4/1
  Add3/1 -> Sat/1(Err_now)
  Constant8/1 -> Sat1/2(h), Sat/2(h)
  Constant9/1 -> Sat1/3(ErrMax), Sat/3(ErrMax)
  Add7/1 -> Sat1/1(Err_now)
  Sat/1(AlphaE) -> Scope2/1, Scope3/1, LPF/1(In), Delay2/1  "AlphaE"
  Delay2/1 -> Add/2
  Sat1/1(AlphaE) -> Scope2/2, Scope4/1, LPF1/1(In), Delay3/1  "BetaE"
  Delay3/1 -> Add4/2
  Constant10/1 -> LPF/2(TiCon), LPF1/2(TiCon)
  LPF/1(out) -> Scope3/2, AlphaE/1
  LPF1/1(out) -> Scope4/2, BetaE/1

== system PMSM_MC_2025a/PMSM_MC/MC_HighFrqTask/FOC/SensorLessAlgorithm/FluxObs+PLL/PLL/LPF ==
  In : Inport
  TiCon : Inport  Port=2
  Add : Sum  Inputs=+-
  Add1 : Sum
  Constant : Constant  Value=single(1)
  Delay : Delay  DelayLength=1  InitialConditionSource=Input port
      settings: InputPortMap=u0,p4
  Product : Product
  Product1 : Product
  out : Outport
  wires:
  Delay/1 -> Product1/2
  Add1/1 -> out/1, Delay/1
  Product1/1 -> Add1/2
  Product/1 -> Add1/1
  Constant/1 -> Add/1
  Add/1 -> Product1/1
  TiCon/1 -> Product/2, Add/2
  In/1 -> Product/1, Delay/2

== system PMSM_MC_2025a/PMSM_MC/MC_HighFrqTask/FOC/SensorLessAlgorithm/Luenberger+PLL/Luenberger/LPF ==
  In : Inport
  TiCon : Inport  Port=2
  Add : Sum  Inputs=+-
  Add1 : Sum
  Constant : Constant  Value=single(1)
  Delay : Delay  DelayLength=1  InitialConditionSource=Input port
      settings: InputPortMap=u0,p4
  Product : Product
  Product1 : Product
  out : Outport
  wires:
  Delay/1 -> Product1/2
  Add1/1 -> out/1, Delay/1
  Product1/1 -> Add1/2
  Product/1 -> Add1/1
  Constant/1 -> Add/1
  Add/1 -> Product1/1
  TiCon/1 -> Product/2, Add/2
  In/1 -> Product/1, Delay/2

== system PMSM_MC_2025a/PMSM_MC/MC_HighFrqTask/FOC/SensorLessAlgorithm/Luenberger+PLL/Luenberger/LPF1 ==
  In : Inport
  TiCon : Inport  Port=2
  Add : Sum  Inputs=+-
  Add1 : Sum
  Constant : Constant  Value=single(1)
  Delay : Delay  DelayLength=1  InitialConditionSource=Input port
      settings: InputPortMap=u0,p4
  Product : Product
  Product1 : Product
  out : Outport
  wires:
  In/1 -> Delay/2, Product/1
  TiCon/1 -> Add/2, Product/2
  Add/1 -> Product1/1
  Constant/1 -> Add/1
  Product/1 -> Add1/1
  Product1/1 -> Add1/2
  Add1/1 -> Delay/1, out/1
  Delay/1 -> Product1/2

== system PMSM_MC_2025a/PMSM_MC/MC_HighFrqTask/FOC/SensorLessAlgorithm/Luenberger+PLL/PLL/LPF ==
  In : Inport
  TiCon : Inport  Port=2
  Add : Sum  Inputs=+-
  Add1 : Sum
  Constant : Constant  Value=single(1)
  Delay : Delay  DelayLength=1  InitialConditionSource=Input port
      settings: InputPortMap=u0,p4
  Product : Product
  Product1 : Product
  out : Outport
  wires:
  In/1 -> Delay/2, Product/1
  TiCon/1 -> Add/2, Product/2
  Add/1 -> Product1/1
  Constant/1 -> Add/1
  Product/1 -> Add1/1
  Product1/1 -> Add1/2
  Add1/1 -> Delay/1, out/1
  Delay/1 -> Product1/2

== system PMSM_MC_2025a/PMSM_MC/MC_HighFrqTask/FOC/SensorLessAlgorithm/SMO+PLL/PLL/LPF ==
  In : Inport
  TiCon : Inport  Port=2
  Add : Sum  Inputs=+-
  Add1 : Sum
  Constant : Constant  Value=single(1)
  Delay : Delay  DelayLength=1  InitialConditionSource=Input port
      settings: InputPortMap=u0,p4
  Product : Product
  Product1 : Product
  out : Outport
  wires:
  In/1 -> Delay/2, Product/1
  TiCon/1 -> Add/2, Product/2
  Add/1 -> Product1/1
  Constant/1 -> Add/1
  Product/1 -> Add1/1
  Product1/1 -> Add1/2
  Add1/1 -> Delay/1, out/1
  Delay/1 -> Product1/2

== system PMSM_MC_2025a/PMSM_MC/MC_HighFrqTask/FOC/SensorLessAlgorithm/SMO+PLL/SMO/LPF ==
  In : Inport
  TiCon : Inport  Port=2
  Add : Sum  Inputs=+-
  Add1 : Sum
  Constant : Constant  Value=single(1)
  Delay : Delay  DelayLength=1  InitialConditionSource=Input port
      settings: InputPortMap=u0,p4
  Product : Product
  Product1 : Product
  out : Outport
  wires:
  In/1 -> Delay/2, Product/1
  TiCon/1 -> Add/2, Product/2
  Add/1 -> Product1/1
  Constant/1 -> Add/1
  Product/1 -> Add1/1
  Product1/1 -> Add1/2
  Add1/1 -> Delay/1, out/1
  Delay/1 -> Product1/2

== system PMSM_MC_2025a/PMSM_MC/MC_HighFrqTask/FOC/SensorLessAlgorithm/SMO+PLL/SMO/LPF1 ==
  In : Inport
  TiCon : Inport  Port=2
  Add : Sum  Inputs=+-
  Add1 : Sum
  Constant : Constant  Value=single(1)
  Delay : Delay  DelayLength=1  InitialConditionSource=Input port
      settings: InputPortMap=u0,p4
  Product : Product
  Product1 : Product
  out : Outport
  wires:
  Delay/1 -> Product1/2
  Add1/1 -> out/1, Delay/1
  Product1/1 -> Add1/2
  Product/1 -> Add1/1
  Constant/1 -> Add/1
  Add/1 -> Product1/1
  TiCon/1 -> Product/2, Add/2
  In/1 -> Product/1, Delay/2

== system PMSM_MC_2025a/PMSM_MC/MC_HighFrqTask/FOC/SensorLessAlgorithm/SMO+PLL/SMO/Sat ==
  Err_now : Inport
  h : Inport  Port=2
  ErrMax : Inport  Port=3
  Constant : Constant  Value=single(1)
  Constant1 : Constant  Value=single(-1)
  Divide : Product  Inputs=*/
  Gain : Gain  Gain=-1
  Product : Product
  Relational Operator : RelationalOperator  Operator=>  OutDataTypeStr=boolean  RndMeth=Simplest  InputSameDT=off
  Relational Operator1 : RelationalOperator  Operator=<  OutDataTypeStr=boolean  RndMeth=Simplest  InputSameDT=off
  Switch : Switch  Criteria=u2 ~= 0  SaturateOnIntegerOverflow=off  InputSameDT=off
  Switch1 : Switch  Criteria=u2 ~= 0  SaturateOnIntegerOverflow=off  InputSameDT=off
  AlphaE : Outport
  wires:
  Err_now/1 -> Divide/1, Relational Operator1/1, Relational Operator/1
  ErrMax/1 -> Divide/2, Gain/1, Relational Operator/2
  Relational Operator/1 -> Switch/2
  Constant/1 -> Switch/1
  Gain/1 -> Relational Operator1/2
  Relational Operator1/1 -> Switch1/2
  Switch1/1 -> Switch/3
  Constant1/1 -> Switch1/1
  Divide/1 -> Switch1/3
  Switch/1 -> Product/1
  h/1 -> Product/2
  Product/1 -> AlphaE/1

== system PMSM_MC_2025a/PMSM_MC/MC_HighFrqTask/FOC/SensorLessAlgorithm/SMO+PLL/SMO/Sat1 ==
  Err_now : Inport
  h : Inport  Port=2
  ErrMax : Inport  Port=3
  Constant : Constant  Value=single(1)
  Constant1 : Constant  Value=single(-1)
  Divide : Product  Inputs=*/
  Gain : Gain  Gain=-1
  Product : Product
  Relational Operator : RelationalOperator  Operator=>  OutDataTypeStr=boolean  RndMeth=Simplest  InputSameDT=off
  Relational Operator1 : RelationalOperator  Operator=<  OutDataTypeStr=boolean  RndMeth=Simplest  InputSameDT=off
  Switch : Switch  Criteria=u2 ~= 0  SaturateOnIntegerOverflow=off  InputSameDT=off
  Switch1 : Switch  Criteria=u2 ~= 0  SaturateOnIntegerOverflow=off  InputSameDT=off
  AlphaE : Outport
  wires:
  Err_now/1 -> Divide/1, Relational Operator1/1, Relational Operator/1
  ErrMax/1 -> Divide/2, Gain/1, Relational Operator/2
  Relational Operator/1 -> Switch/2
  Constant/1 -> Switch/1
  Gain/1 -> Relational Operator1/2
  Relational Operator1/1 -> Switch1/2
  Switch1/1 -> Switch/3
  Constant1/1 -> Switch1/1
  Divide/1 -> Switch1/3
  Switch/1 -> Product/1
  h/1 -> Product/2
  Product/1 -> AlphaE/1

== stateflow chart PMSM_MC_2025a/Scheduler ==
  (default) -> (junction 6)
  (junction 6) -> (junction 11) [order 1] : [counter%%20==19]
  (junction 6) -> (junction 10) [order 2]
  (junction 11) -> (junction 9) : {trig_MidFrq_1ms;}
  (junction 9) -> (junction 10)
  (junction 10) -> (junction 18) : {trig_HighFrq_50us;}
  (junction 18) -> (junction 20) [order 1] : [counter>=100000000]
  (junction 18) -> (junction 24) [order 2] : {counter++;}
  (junction 20) -> (junction 22) : {counter=0;}
  (junction 22) -> (junction 24)
  (junction 24) -> (junction 27)
  data: counter local uint32 =0
  events: trig_MidFrq_1ms output FUNCTION_CALL_EVENT; trig_HighFrq_50us output FUNCTION_CALL_EVENT

== stateflow chart PMSM_MC_2025a/PMSM_MC/MC_LowFrqTask/SpdLoop/SensorlessSpeedCtrl ==
  state Stop
    en:
    SpdRef = 0.0F;
    SpdInt = 0.0F;
    IqRef = 0.0F;
    SL_SpeedReady = false;
  state IFCurrent [function]
    (default) -> (junction 23) : {
        | SpdRef = 300.0F;
        | IqRef = 0.6F;
        | }
    (junction 23) -> (junction 26) [order 1] : [MotorSpdRef < 0.0F]
    (junction 23) -> (junction 30) [order 2]
    (junction 26) -> (junction 28) : {
        | SpdRef = -SpdRef;
        | IqRef = -IqRef;
        | }
    (junction 28) -> (junction 30)
    (junction 30) -> (junction 33) : {
        | SpdInt =IqRef - MC_SpdLopKp_CFG * (SpdRef - MotorActSpd);
        | SL_SpeedReady = MotorActSpd > SpdRef - 30.0F && MotorActSpd < SpdRef + 30.0F;
        | }
  state IF
    en,du:
    IFCurrent();
  state Reference [function]
    (default) -> (junction 36)
    (junction 36) -> (junction 37) [order 1] : [MotCtrMode == 7]
    (junction 37) -> (junction 39) [order 1] : [MotorSpdRef<0]
    (junction 36) -> (junction 38) [order 2] : {
        | RawNow = MotorSpdRef - SpdRef;
        | }
    (junction 37) -> (junction 51) [order 2] : {
        | SpdRef = 300.0F;
        | }
    (junction 39) -> (junction 49) : {
        | SpdRef = -300.0F;
        | }
    (junction 49) -> (junction 51)
    (junction 51) -> (junction 147)
    (junction 38) -> (junction 56)
    (junction 56) -> (junction 58) [order 1]
    (junction 58) -> (junction 60) [order 1] : [RawNow > 1.0F]
    (junction 56) -> (junction 69) [order 2] : {
        | SpdRef = MotorSpdRef;
        | }
    (junction 58) -> (junction 66) [order 2] : [RawNow < -1.0F]
    (junction 60) -> (junction 62) : {
        | SpdRef = SpdRef + 1.0F;
        | }
    (junction 66) -> (junction 64) : {
        | SpdRef = SpdRef - 1.0F;
        | }
    (junction 64) -> (junction 69)
    (junction 62) -> (junction 64)
    (junction 147) -> (junction 69)
    (junction 69) -> (junction 72) : {
        | SL_SpeedReady = (MotCtrMode == 7) && MotorActSpd > SpdRef - 30.0F && MotorActSpd < SpdRef + 30.0F;
        | }
  state Run
    en:
    Reference();
    Err = SpdRef - MotorActSpd;
    SpdInt = IqRef - MC_SpdLopKp_CFG * Err;
    SpeedPI();
    du:
    Reference();
    SpeedPI();
  state SpeedPI [function]
    (default) -> (junction 75) : {
        | Err = SpdRef - MotorActSpd;
        | RawNow = MC_SpdLopKp_CFG * Err + SpdInt;
        | }
    (junction 75) -> (junction 107) [order 1]
    (junction 107) -> (junction 109) [order 1] : [RawNow > 3.0F]
    (junction 75) -> (junction 118) [order 2] : {
        | IqRef = RawNow;
        | }
    (junction 107) -> (junction 115) [order 2] : [RawNow < -3.0F]
    (junction 109) -> (junction 111) : {
        | IqRef = 3.0F;
        | }
    (junction 115) -> (junction 113) : {
        | IqRef = -3.0F;
        | }
    (junction 113) -> (junction 118)
    (junction 111) -> (junction 113)
    (junction 118) -> (junction 121)
    (junction 121) -> (junction 123) [order 1] : [!((RawNow >= 3.0F && Err > 0.0F) || (RawNow <= -3.0F && Err < 0.0F))]
    (junction 121) -> (junction 127) [order 2]
    (junction 123) -> (junction 125) : {
        | SpdInt = SpdInt + MC_SpdLopKi_CFG * Err;
        | }
    (junction 125) -> (junction 127)
    (junction 127) -> (junction 134)
    (junction 134) -> (junction 132) [order 1]
    (junction 132) -> (junction 133) [order 1] : [SpdInt > 3.0F]
    (junction 134) -> (junction 142) [order 2]
    (junction 132) -> (junction 130) [order 2] : [SpdInt < -3.0F]
    (junction 133) -> (junction 137) : {
        | SpdInt = 3.0F;
        | }
    (junction 130) -> (junction 135) : {
        | SpdInt = -3.0F;
        | }
    (junction 135) -> (junction 142)
    (junction 137) -> (junction 135)
  (default) -> Stop
  Stop -> IF : [MotCtrMode == 7]
  IF -> Stop [order 2] : [MotCtrMode != 7 && MotCtrMode != 5]
  Run -> Stop : [MotCtrMode != 7 && MotCtrMode != 5]
  IF -> Run [order 1] : [SL_TransferActive || MotCtrMode == 5]
  data: MotCtrMode input uint8; MotorSpdRef input single; MotorActSpd input single; IqRef output single; SL_TransferActive data_store_memory; SL_SpeedReady data_store_memory; MC_SpdLopKp_CFG parameter single; MC_SpdLopKi_CFG parameter single; SpdRef local single; SpdInt local single; Err local single; RawNow local single

== stateflow chart PMSM_MC_2025a/PMSM_MC/MC_LowFrqTask/MotModeCtr/ModeMgr ==
  state RangeCheck [function]
    (default) -> (junction 21)
    (junction 21) -> (junction 23) [order 1] : [abs(MotOffsetBuff[0]-MotOffsetBuff[1])>100]
    (junction 21) -> (junction 24) [order 2] : {
        | MotCalNormal=1;
        | MotOffset = (MotOffsetBuff[0]+MotOffsetBuff[1])/2;
        | }
    (junction 23) -> (junction 25) : {MotCalNormal=0;}
    (junction 25) -> (junction 24)
    (junction 24) -> (junction 35)
  state SensorCtr
    state Calibrate
      state Init
        en:
        MotCtrMode=0;
      state Calibrate1
        en:
        MotCtrMode=1;
        MotCalThetae = 0;//0°
      state Calibrate2
        en:
        MotOffsetBuff[0]=Ecode_cnt;
        MotCtrMode=2;
        MotCalThetae = 0;//0°
      state RngChk
        en:
        MotOffsetBuff[1]=Ecode_cnt;
        RangeCheck();
      (default) -> Init
      Init -> Calibrate1 : [MotorSpdRef != 0]
      Calibrate1 -> Calibrate2 : [after(1.5,sec)]
      Calibrate2 -> RngChk : [after(1.5,sec)]
    state Normal
      state Stop
        en:
        MotCtrMode=4;
      state Run
        en:
        MotCtrMode=5;
      (default) -> SensorCtr.Normal.Stop
      SensorCtr.Normal.Run -> SensorCtr.Normal.Stop : [MotorSpdRef==0]
      SensorCtr.Normal.Stop -> SensorCtr.Normal.Run : [MotorSpdRef!=0]
    state CalFailed
      en:
      MotCtrMode=3;
    (default) -> Calibrate
    CalFailed -> Calibrate : [MotorSpdRef==0]
    RngChk -> CalFailed [order 1] : [MotCalNormal==0]
    RngChk -> Normal [order 2] : [MotCalNormal==1]
  state SensorLessCtr
    state Stop
      en:
      MotCtrMode=4;
    state StartFail
      en:
      MotCtrMode=6;
    state IFStart
      en:
      MotCtrMode=7;
    state Run
      en:
      MotCtrMode=5;
    (default) -> SensorLessCtr.Stop
    SensorLessCtr.Stop -> IFStart : [MotorSpdRef != 0]
    StartFail -> SensorLessCtr.Stop : [MotorSpdRef==0]
    SensorLessCtr.Run -> SensorLessCtr.Stop : [MotorSpdRef==0]
    IFStart -> StartFail [order 2] : [after(10.0,sec)]
    IFStart -> SensorLessCtr.Run [order 1] : [OLStartCompletedFlag==1]
  note: 注意此处的无感有感开环状态机
      | 的切换模式条件中，如果是仿真
      | 测试需要把速度设定改成不等于
      | 0，但是嵌入式模型部署中需要
      | 改成等于0
  state VFOpenLoop
    en:
    MotCtrMode = 8;
  (default) -> SensorCtr
  SensorCtr -> SensorLessCtr [order 1] : [//value is 1 mean sensorless control
      | SensorLessEn ==1 &&...
      | MotorSpdRef != 0]
  SensorLessCtr -> SensorCtr [order 1] : [//value is 0 mean sensor control
      | SensorLessEn ==0 &&...
      | MotorSpdRef != 0]
  SensorLessCtr -> VFOpenLoop [order 2] : [OpenLoopEn == 1&&...
      | MotorSpdRef != 0]
  VFOpenLoop -> SensorLessCtr [order 1] : [OpenLoopEn == 0&&...
      | MotorSpdRef != 0&&...
      | SensorLessEn == 1]
  VFOpenLoop -> SensorCtr [order 2] : [OpenLoopEn == 0&&...
      | MotorSpdRef != 0&&...
      | SensorLessEn == 0]
  SensorCtr -> VFOpenLoop [order 2] : [OpenLoopEn == 1&&...
      | MotorSpdRef != 0]
  data: MotCtrMode output uint8; Ecode_cnt input int32; MotorSpdRef input int16; MotOffset output int32; MotCalThetae output single; MotOffsetBuff local int32 size=2; MotCalNormal local boolean; SensorLessEn input boolean; OpenLoopEn input boolean; OLStartCompletedFlag input boolean
